simulink subsystem "swingup_energy"  (R2023a)
settings: Solver=VariableStepAuto  StartTime=0.0  StopTime=10.0  RelTol=1e-3
settings Model: Creator=ahmad  LastModifiedBy=ahmad
settings ModelReferenceCC: UpdateModelReferenceTargets=IfOutOfDate
settings RTWCC: GPUComputeCapability=5.0
settings ConfigComp: CovBoundaryAbsTol=1.0e-5

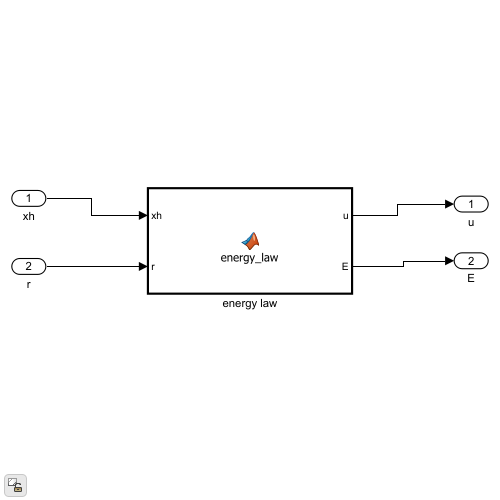
[thumbnail: Simulink's stored preview of the top-level diagram]
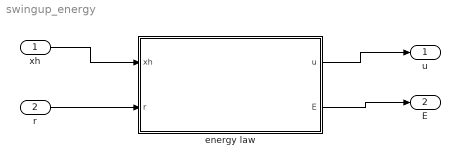
== system swingup_energy ==
  xh : Inport  PortDimensions=4
  r : Inport  Port=2
  energy law : MATLAB Function  TreatAsAtomicUnit=on
  u : Outport
  E : Outport  Port=2
  wires:
  xh/1 -> energy law/1(xh)
  r/1 -> energy law/2(r)
  energy law/1(u) -> u/1
  energy law/2(E) -> E/1

== matlab function swingup_energy/energy law ==
  data: xh input; u output; r input; E output; ctrlP parameter
function [u, E] = energy_law(xh, r, ctrlP)
% Energy swing-up (report section 10). Knobs: ctrlP.swing (ctrl_hybrid_design.m, swingup_knobs.m).
% Inputs: xh = [th0; th1 (0 up, wrapped); w0; w1], r = arm reference. Outputs: duty u, energy E.
% Pendulum energy in the report's scaled units (eq. 89): 0 at rest upright, -2G hanging.
m = ctrlP.plant;
s = ctrlP.swing;
th0 = xh(1); th1 = xh(2); w0 = xh(3); w1 = xh(4);
E = 0.5*m.Jp*w1^2 + m.G*(cos(th1) - 1);
e = E/(2*m.G);                                  % -1 hanging still, 0 just reaches the top

% 1. pump: accelerate the pivot against the bob, dE/dt = -h cos(th1) w1 a0. Full size until
%    close to the target E0 (slightly above the top), then fades; above E0 it brakes.
a0 = -s.a_push*min(1, max(-1, s.k_E*(s.E0 - e)))*tanh(w1*cos(th1)/s.w_sign);

% 2. kick: a still, hanging pendulum gives no direction to push in -> push the arm once.
if e < -1 + s.kick_E
    a0 = s.a_kick;
end

% 3. soft spring and damper that keep the arm near its reference.
a0 = a0 - s.wc^2*(th0 - r) - 2*s.zc*s.wc*w0;

% 4. acceleration -> motor current (arm inertia, viscous and dry friction), limited;
%    -> duty with the back-EMF added, so the current stays at the command even when reversing.
%    Dry friction: the sliding Coulomb friction; with the arm at rest it blends to the breakaway
%    (13 % / 14 % duty, measured) in the direction of the wanted acceleration (firmware 1.8). Without
%    it the kick from rest asked for 11 % duty and the arm never moved on the rig. stick_gain 0 = off.
sf = tanh(w0/s.w_fric);
coul = m.tcp*max(sf, 0) + m.tcn*min(sf, 0);
sa = tanh(a0/s.a_stick);
stat = m.tsp*max(sa, 0) + m.tsn*min(sa, 0);
g = exp(-(w0/s.w_stick)^2);
i = m.Ja*a0 + m.Beq*w0 + coul + s.stick_gain*g*(stat - coul);
i = min(s.i_max, max(-s.i_max, i));
u = (m.Rm*i + m.Kb*w0)/m.Vs;
u = min(s.u_max, max(-s.u_max, u));
